simulink model "Pierre_Controller_LTI_2026b"  (R2025b)
settings: Solver=ode1  StartTime=0.0  StopTime=inf  FixedStep=Ts  RelTol=1e-3
PostLoadFcn:
  | , if any(exist('dsrtsu_mdlpostloadfcn', 'file') ~= 0), dsrtsu_mdlpostloadfcn('Execute', bdroot); end,
InitFcn:
  | , if any(exist('rtifpga_mdlclblib', 'file') ~= 0), rtifpga_mdlclblib('Init', bdroot); end,
values from neighbouring files (symbols this model uses):
  BUTTER = ss(A,B,C,D,Ts)    [build_model.m]
  K = opensave.K_final    [build_model.m]
  Px = 1    [build_model.m]
  Py = 1    [build_model.m]
  Pz = 1    [build_model.m]
  S_Sensor = 0.1134    [build_model.m]
  Sen_AX = 2.0176    [build_model.m]
  Sen_AY = 2.011    [build_model.m]
  Sen_AZ = 2.0066    [build_model.m]
  Sen_GX = 0.75481    [build_model.m]
  Sen_GY = 0.75728    [build_model.m]
  Sen_GZ = 0.74931    [build_model.m]
  Sweep_amp = 0.5    [build_model.m]
  Switch_excit = 4    [build_model.m]
  TMS_amp = 2    [build_model.m]
  TMS_freq1 = 80    [build_model.m]
  TMS_freq2 = 0    [build_model.m]
  TMS_freq3 = 0    [build_model.m]
  Ts = 1/Fs    (= 0.001)    [build_model.m]
  V_sat = 2/10    (= 0.2)    [build_model.m]
  V_sat_TMS = 5    [build_model.m]
undefined symbols (not defined in the file or in its folder): R, S
libraries: dspfdesign x15, rti1202lib_adc_class1 x10, rti1202lib_dac_class1 x7, rti1202lib_adc_class2 x6, dspxfrm3 x3, cstblocks x1, simulink x1
(part 1 of 3)
PreSaveFcn:
  | , if any(exist('dsmpb_private', 'file') == [2, 3, 6]), try, dsmpb_private('dsmpb_mdlclblib', 'PreSave', bdroot); catch, disp(lasterr); end, end,
CloseFcn:
  | , if any(exist('dsmpb_private', 'file') == [2, 3, 6]), try, dsmpb_private('dsmpb_mdlclblib', 'Close', bdroot); catch, disp(lasterr); end, end,
settings Model: DSRTSU_INTERNAL_RTI_VER=670  DSRTSU_INTERNAL_RTI_TYPE=rti1202  RTICANMMDATA=struct('GeneralSetupData',struct('modelroot','C:\PROJECTS\OSIP_VIB\Simulink\Feedback_LTI','generalsettings',struct('filesettings',struct('destfolder',struct('Name','RTICANMM_FILES','Check',1),'buildfolder',struct('Name','.','Check',1),'AbsDestfolder',struct('Name','C:\PROJECTS\OSIP_VIB\Simulink\Feedback_LTI\RTICANMM_FILES'),'AbsBuildfolder',struct('Name','C:\PROJECTS\OSIP_VIB\Simulink\Feedback_LTI'))),'options',struct('addpaths',1,'rmpaths',1,'addtrcexclusion',logical(1),'cannavigator',struct('checkmonitoring',0),'show_usrtrc',0,'use_usrtrc',0),'advanced',struct('options',[1 1 1 1 1 1 1 1 1 1 1 1 1 1 1 1 1 1 1 1 1 1 1 1 1 1 1 1 1 1 1 1 1 1 1 1 1 1 1 1 1 1 1 1 1 1 1 1 1 1 1 1 1 1 1 1 1 1 1 1 1 1 1 1 1 1 1 1 1 1 1 1 1 1 1 1 1 1 1 1 1 1 1 1 1 1 1 1 1 1 1 1 1 1 1 1 1 1 1 1]),'MPSetup',{{}},'modelname','Feedback_LTI','block','Feedback_LTI'))  DSRTSU_INTERNAL_RTIFPGA=231  DSMPB_DATASERVER_ModelPortLibVersion1=8  DSMPB_DATASERVER_DataServerVersion1=6  DSMPB_DATASERVER_DataServerStreamVersion1=3  DSRTSU_INTERNAL_RTISTBM_VER=25.2  Creator=yjr  LastModifiedBy=pgr
settings SolverCC: AlgebraicLoopSolver=TrustRegion
settings OptimizationCC: BlockReduction=off  OptimizeBlockIOStorage=off  BufferReuse=off  GlobalBufferReuse=off  ExpressionFolding=off  LocalBlockOutputs=off
settings DebuggingCC: UnconnectedInputMsg=warning  UnconnectedOutputMsg=warning  UnconnectedLineMsg=warning  ArithmeticOperatorsInVariantConditions=warning
settings HardwareCC: ProdBitPerPointer=32.0  ProdBitPerSizeT=32.0  ProdBitPerPtrDiffT=32.0  ProdLargestAtomicInteger=Integer  ProdEndianess=BigEndian  ProdWordSize=32.0  ProdHWDeviceType=Custom Processor->Custom  TargetIntDivRoundTo=Zero  TargetEndianess=BigEndian  TargetHWDeviceType=Custom Processor->Custom
settings ModelReferenceCC: EnableRefExpFcnMdlSchedulingChecks=on
settings SFSimCC: SimUseLocalCustomCode=off  MATLABDynamicMemAlloc=off  CustomCodeUndefinedFunction=UseInterfaceOnly
settings RTWCC: SystemTargetFile=rti1202.tlc  GenCodeOnly=on  MakeCommand=make_rti  TemplateMakefile=rti1202.tmf  RTWUseLocalCustomCode=off  GPUComputeCapability=3.5  Description=dSPACE DS1202 Hardware Platform
settings CodeAppCC: StateflowObjectComments=on
settings STFCustomTargetCC: SystemTargetFile=rti1202.tlc  ParMdlRefBuildCompliant=on  ConcurrentExecutionCompliant=off  GRTInterface=off  InitialSimState=RUN  LoadAfterBuild=off  TRCOnlyGlobals=off  EnableRealTimeTesting=on  BoardName=ds1202  TRCGenerateDerivatives=off  ExecutionMode=real-time  LoadApplNonUI=OFF  PlatformSelectionPopup=Platform Name  RTICfgSetVer=670.0  NISValue=1  NetworkClientNonUI=OPTION_DISABLED  TRCGenerateStates=off  CCompilerOptimizationOptsNonUI=USE_DEFAULT  TRCGenerateLabels=off  LoadToFlash=off  AllowReservedHostServiceNums=off  TimeScaleFactor=1.0  AssertionMode=OFF  TRCIsOmitVdOn=off  EnableRealTimeTestingNonUI=ON  ExecutionModeNonUI=RTSIM  VDFType=TRC  CCompilerOptimizationOptsPopup_=Default  FSIValue=0  TaskModeNonUI=LOW_JITTER  TRCGenerateVirtualBlocks=off  BoardNameNonUI=ds1202  TimeScaleFactorNonUI=OPTION_DISABLED  TaskMode=Low jitter, low latency tasks  TRCGenerateParamValues=on
settings GRTTargetCC: TargetLangStandard=C89/C90 (ANSI)  CompOptLevelCompliant=off  ConcurrentExecutionCompliant=off  CombineOutputUpdateFcns=off  MatFileLogging=off  CPPClassGenCompliant=off  UseToolchainInfoCompliant=off
settings ConfigComp: CovMetricSettings=dswe

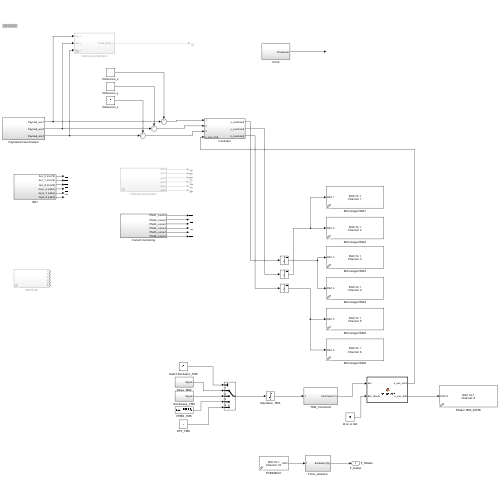
[thumbnail: Simulink's stored preview of the top-level diagram]
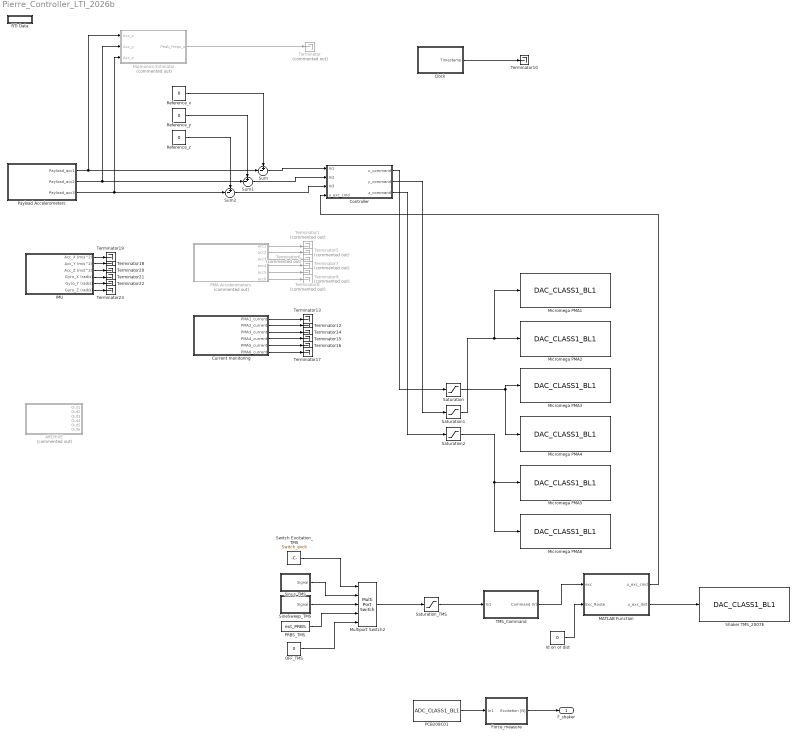
== system Pierre_Controller_LTI_2026b ==
  ARCHIVE : Subsystem  Commented=on
  Clock : Subsystem
  Controller : Subsystem
  Current monitoring : Subsystem
  Force_measure : Subsystem
  Harmonics Estimator : Subsystem  Commented=on
  IMU : Subsystem
  Id on or dist : Constant  Value=0
  MATLAB Function : MATLAB Function  TreatAsAtomicUnit=on
  Micromega PMA1 : rti1202lib_dac_class1/DAC_CLASS1_BL1  DSProperties=struct('RTI',struct('Version',uint32(2),'BlockType',struct('isSLSource',uint8(0),'isSLSink',uint8(1),'isHWSource',uint8(0),'isHWSink',uint8(1),'isSetup',uint8(0),'isInline',uint8(1),'isNonInline',uint8(0),'isInterrupt',uint8(0),'isChannelwise',uint8(1)),'IOBoardType',{{'DS120X','STD','DACC1'}},'UnitType','DAC','Identifier','DAC','DialogType','ML','BlockSet','NONE','SlaveProcessor','NONE'))  RTIBlockInterface=struct('InputPortsActive',1,'InputPortsWidth',int32(1),'InputPortsDataType',{{'SS_DOUBLE'}},'InputPortsName',{{['DAC 1']}},'DialogFcn','rti120xstddacc1dacgui','InitLevel',3,'IconTransparency','on','BlockDisplay',{{['DAC CL1\nChannel: 1'],'center'}},'BlockName',struct('Token',{{'DAC_CLASS1_BL1'}}))  RTIBlockParameters=struct('ChannelNo',{{1,'OFF',[]}},'ChannelNumOf',{{1,'OFF',[]}},'InitialValue1',{{0,'OFF',[-10 10]}},'InitialValue2',{{0,'OFF',[-10 10]}},'InitialValue3',{{0,'OFF',[-10 10]}},'InitialValue4',{{0,'OFF',[-10 10]}},'InitialValue5',{{0,'OFF',[-10 10]}},'InitialValue6',{{0,'OFF',[-10 10]}},'InitialValue7',{{0,'OFF',[-10 10]}},'InitialValue8',{{0,'OFF',[-10 10]}},'InitialValue9',{{0,'OFF',[-10 10]}},'InitialValue10',{{0,'OFF',[-10 10]}},'InitialValue11',{{0,'OFF',[-10 10]}},'InitialValue12',{{0,'OFF',[-10 10]}},'InitialValue13',{{0,'OFF',[-10 10]}},'InitialValue14',{{0,'OFF',[-10 10]}},'InitialValue15',{{0,'OFF',[-10 10]}},'InitialValue16',{{0,'OFF',[-10 10]}},'OutputMode',{{ones(1,16),'OFF',[1 2]}},'TermValue1',{{0,'OFF',[-10 10]}},'TermValue2',{{0,'OFF',[-10 10]}},'TermValue3',{{0,'OFF',[-10 10]}},'TermValue4',{{0,'OFF',[-10 10]}},'TermValue5',{{0,'OFF',[-10 10]}},'TermValue6',{{0,'OFF',[-10 10]}},'TermValue7',{{0,'OFF',[-10 10]}},'TermValue8',{{0,'OFF',[-10 10]}},'TermValue9',{{0,'OFF',[-10 10]}},'TermValue10',{{0,'OFF',[-10 10]}},'TermValue11',{{0,'OFF',[-10 10]}},'TermValue12',{{0,'OFF',[-10 10]}},'TermValue13',{{0,'OFF',[-10 10]}},'TermValue14',{{0,'OFF',[-10 10]}},'TermValue15',{{0,'OFF',[-10 10]}},'TermValue16',{{0,'OFF',[-10 10]}},'EnableTermMode',{{0,'OFF',[0 1]}},'TLCFileName',{{'rti120xdac_c1_dac','OFF',[]}},'InitialValueBuildCheck1',{{0,'OFF',[]}},'InitialValueBuildCheck2',{{0,'OFF',[]}},'InitialValueBuildCheck3',{{0,'OFF',[]}},'InitialValueBuildCheck4',{{0,'OFF',[]}},'InitialValueBuildCheck5',{{0,'OFF',[]}},'InitialValueBuildCheck6',{{0,'OFF',[]}},'InitialValueBuildCheck7',{{0,'OFF',[]}},'InitialValueBuildCheck8',{{0,'OFF',[]}},'InitialValueBuildCheck9',{{0,'OFF',[]}},'InitialValueBuildCheck10',{{0,'OFF',[]}},'InitialValueBuildCheck11',{{0,'OFF',[]}},'InitialValueBuildCheck12',{{0,'OFF',[]}},'InitialValueBuildCheck13',{{0,'OFF',[]}},'InitialValueBuildCheck14',{{0,'OFF',[]}},'InitialValueBuildCheck15',{{0,'OFF',[]}},'InitialValueBuildCheck16',{{0,'OFF',[]}},'TermValueBuildCheck1',{{0,'OFF',[]}},'TermValueBuildCheck2',{{0,'OFF',[]}},'TermValueBuildCheck3',{{0,'OFF',[]}},'TermValueBuildCheck4',{{0,'OFF',[]}},'TermValueBuildCheck5',{{0,'OFF',[]}},'TermValueBuildCheck6',{{0,'OFF',[]}},'TermValueBuildCheck7',{{0,'OFF',[]}},'TermValueBuildCheck8',{{0,'OFF',[]}},'TermValueBuildCheck9',{{0,'OFF',[]}},'TermValueBuildCheck10',{{0,'OFF',[]}},'TermValueBuildCheck11',{{0,'OFF',[]}},'TermValueBuildCheck12',{{0,'OFF',[]}},'TermValueBuildCheck13',{{0,'OFF',[]}},'TermValueBuildCheck14',{{0,'OFF',[]}},'TermValueBuildCheck15',{{0,'OFF',[]}},'TermValueBuildCheck16',{{0,'OFF',[]}})  RTISFcnParameters=struct('ChannelNo','int16','ChannelNumOf','int16','InitialValue1','double','InitialValue2','double','InitialValue3','double','InitialValue4','double','InitialValue5','double','InitialValue6','double','InitialValue7','double','InitialValue8','double','InitialValue9','double','InitialValue10','double','InitialValue11','double','InitialValue12','double','InitialValue13','double','InitialValue14','double','InitialValue15','double','InitialValue16','double','OutputMode','int16','TermValue1','double','TermValue2','double','TermValue3','double','TermValue4','double','TermValue5','double','TermValue6','double','TermValue7','double','TermValue8','double','TermValue9','double','TermValue10','double','TermValue11','double','TermValue12','double','TermValue13','double','TermValue14','double','TermValue15','double','TermValue16','double','EnableTermMode','int16','TLCFileName','char')  RTIBlockParaDefault=struct('ChannelNo',1,'ChannelNumOf',1,'InitialValue1',0,'InitialValue2',0,'InitialValue3',0,'InitialValue4',0,'InitialValue5',0,'InitialValue6',0,'InitialValue7',0,'InitialValue8',0,'InitialValue9',0,'InitialValue10',0,'InitialValue11',0,'InitialValue12',0,'InitialValue13',0,'InitialValue14',0,'InitialValue15',0,'InitialValue16',0,'OutputMode',ones(1,16),'TermValue1',0,'TermValue2',0,'TermValue3',0,'TermValue4',0,'TermValue5',0,'TermValue6',0,'TermValue7',0,'TermValue8',0,'TermValue9',0,'TermValue10',0,'TermValue11',0,'TermValue12',0,'TermValue13',0,'TermValue14',0,'TermValue15',0,'TermValue16',0,'EnableTermMode',0,'TLCFileName','rti120xdac_c1_dac','InitialValueBuildCheck1',0,'InitialValueBuildCheck2',0,'InitialValueBuildCheck3',0,'InitialValueBuildCheck4',0,'InitialValueBuildCheck5',0,'InitialValueBuildCheck6',0,'InitialValueBuildCheck7',0,'InitialValueBuildCheck8',0,'InitialValueBuildCheck9',0,'InitialValueBuildCheck10',0,'InitialValueBuildCheck11',0,'InitialValueBuildCheck12',0,'InitialValueBuildCheck13',0,'InitialValueBuildCheck14',0,'InitialValueBuildCheck15',0,'InitialValueBuildCheck16',0,'TermValueBuildCheck1',0,'TermValueBuildCheck2',0,'TermValueBuildCheck3',0,'TermValueBuildCheck4',0,'TermValueBuildCheck5',0,'TermValueBuildCheck6',0,'TermValueBuildCheck7',0,'TermValueBuildCheck8',0,'TermValueBuildCheck9',0,'TermValueBuildCheck10',0,'TermValueBuildCheck11',0,'TermValueBuildCheck12',0,'TermValueBuildCheck13',0,'TermValueBuildCheck14',0,'TermValueBuildCheck15',0,'TermValueBuildCheck16',0)
  Micromega PMA2 : rti1202lib_dac_class1/DAC_CLASS1_BL1  DSProperties=struct('RTI',struct('Version',uint32(2),'BlockType',struct('isSLSource',uint8(0),'isSLSink',uint8(1),'isHWSource',uint8(0),'isHWSink',uint8(1),'isSetup',uint8(0),'isInline',uint8(1),'isNonInline',uint8(0),'isInterrupt',uint8(0),'isChannelwise',uint8(1)),'IOBoardType',{{'DS120X','STD','DACC1'}},'UnitType','DAC','Identifier','DAC','DialogType','ML','BlockSet','NONE','SlaveProcessor','NONE'))  RTIBlockInterface=struct('InputPortsActive',1,'InputPortsWidth',int32(1),'InputPortsDataType',{{'SS_DOUBLE'}},'InputPortsName',{{['DAC 2']}},'DialogFcn','rti120xstddacc1dacgui','InitLevel',3,'IconTransparency','on','BlockDisplay',{{['DAC CL1\nChannel: 2'],'center'}},'BlockName',struct('Token',{{'DAC_CLASS1_BL1'}}))  RTIBlockParameters=struct('ChannelNo',{{2,'OFF',[]}},'ChannelNumOf',{{1,'OFF',[]}},'InitialValue1',{{'0','OFF',[-10 10]}},'InitialValue2',{{'0','OFF',[-10 10]}},'InitialValue3',{{'0','OFF',[-10 10]}},'InitialValue4',{{'0','OFF',[-10 10]}},'InitialValue5',{{'0','OFF',[-10 10]}},'InitialValue6',{{'0','OFF',[-10 10]}},'InitialValue7',{{'0','OFF',[-10 10]}},'InitialValue8',{{'0','OFF',[-10 10]}},'InitialValue9',{{'0','OFF',[-10 10]}},'InitialValue10',{{'0','OFF',[-10 10]}},'InitialValue11',{{'0','OFF',[-10 10]}},'InitialValue12',{{'0','OFF',[-10 10]}},'InitialValue13',{{'0','OFF',[-10 10]}},'InitialValue14',{{'0','OFF',[-10 10]}},'InitialValue15',{{'0','OFF',[-10 10]}},'InitialValue16',{{'0','OFF',[-10 10]}},'OutputMode',{{ones(1,16),'OFF',[1 2]}},'TermValue1',{{'0','OFF',[-10 10]}},'TermValue2',{{'0','OFF',[-10 10]}},'TermValue3',{{'0','OFF',[-10 10]}},'TermValue4',{{'0','OFF',[-10 10]}},'TermValue5',{{'0','OFF',[-10 10]}},'TermValue6',{{'0','OFF',[-10 10]}},'TermValue7',{{'0','OFF',[-10 10]}},'TermValue8',{{'0','OFF',[-10 10]}},'TermValue9',{{'0','OFF',[-10 10]}},'TermValue10',{{'0','OFF',[-10 10]}},'TermValue11',{{'0','OFF',[-10 10]}},'TermValue12',{{'0','OFF',[-10 10]}},'TermValue13',{{'0','OFF',[-10 10]}},'TermValue14',{{'0','OFF',[-10 10]}},'TermValue15',{{'0','OFF',[-10 10]}},'TermValue16',{{'0','OFF',[-10 10]}},'EnableTermMode',{{0,'OFF',[0 1]}},'TLCFileName',{{'rti120xdac_c1_dac','OFF',[]}},'InitialValueBuildCheck1',{{0,'OFF',[]}},'InitialValueBuildCheck2',{{1,'OFF',[]}},'InitialValueBuildCheck3',{{0,'OFF',[]}},'InitialValueBuildCheck4',{{0,'OFF',[]}},'InitialValueBuildCheck5',{{0,'OFF',[]}},'InitialValueBuildCheck6',{{0,'OFF',[]}},'InitialValueBuildCheck7',{{0,'OFF',[]}},'InitialValueBuildCheck8',{{0,'OFF',[]}},'InitialValueBuildCheck9',{{0,'OFF',[]}},'InitialValueBuildCheck10',{{0,'OFF',[]}},'InitialValueBuildCheck11',{{0,'OFF',[]}},'InitialValueBuildCheck12',{{0,'OFF',[]}},'InitialValueBuildCheck13',{{0,'OFF',[]}},'InitialValueBuildCheck14',{{0,'OFF',[]}},'InitialValueBuildCheck15',{{0,'OFF',[]}},'InitialValueBuildCheck16',{{0,'OFF',[]}},'TermValueBuildCheck1',{{0,'OFF',[]}},'TermValueBuildCheck2',{{0,'OFF',[]}},'TermValueBuildCheck3',{{0,'OFF',[]}},'TermValueBuildCheck4',{{0,'OFF',[]}},'TermValueBuildCheck5',{{0,'OFF',[]}},'TermValueBuildCheck6',{{0,'OFF',[]}},'TermValueBuildCheck7',{{0,'OFF',[]}},'TermValueBuildCheck8',{{0,'OFF',[]}},'TermValueBuildCheck9',{{0,'OFF',[]}},'TermValueBuildCheck10',{{0,'OFF',[]}},'TermValueBuildCheck11',{{0,'OFF',[]}},'TermValueBuildCheck12',{{0,'OFF',[]}},'TermValueBuildCheck13',{{0,'OFF',[]}},'TermValueBuildCheck14',{{0,'OFF',[]}},'TermValueBuildCheck15',{{0,'OFF',[]}},'TermValueBuildCheck16',{{0,'OFF',[]}})  RTISFcnParameters=struct('ChannelNo','int16','ChannelNumOf','int16','InitialValue1','double','InitialValue2','double','InitialValue3','double','InitialValue4','double','InitialValue5','double','InitialValue6','double','InitialValue7','double','InitialValue8','double','InitialValue9','double','InitialValue10','double','InitialValue11','double','InitialValue12','double','InitialValue13','double','InitialValue14','double','InitialValue15','double','InitialValue16','double','OutputMode','int16','TermValue1','double','TermValue2','double','TermValue3','double','TermValue4','double','TermValue5','double','TermValue6','double','TermValue7','double','TermValue8','double','TermValue9','double','TermValue10','double','TermValue11','double','TermValue12','double','TermValue13','double','TermValue14','double','TermValue15','double','TermValue16','double','EnableTermMode','int16','TLCFileName','char')  RTIBlockParaDefault=struct('ChannelNo',1,'ChannelNumOf',1,'InitialValue1',0,'InitialValue2',0,'InitialValue3',0,'InitialValue4',0,'InitialValue5',0,'InitialValue6',0,'InitialValue7',0,'InitialValue8',0,'InitialValue9',0,'InitialValue10',0,'InitialValue11',0,'InitialValue12',0,'InitialValue13',0,'InitialValue14',0,'InitialValue15',0,'InitialValue16',0,'OutputMode',ones(1,16),'TermValue1',0,'TermValue2',0,'TermValue3',0,'TermValue4',0,'TermValue5',0,'TermValue6',0,'TermValue7',0,'TermValue8',0,'TermValue9',0,'TermValue10',0,'TermValue11',0,'TermValue12',0,'TermValue13',0,'TermValue14',0,'TermValue15',0,'TermValue16',0,'EnableTermMode',0,'TLCFileName','rti120xdac_c1_dac','InitialValueBuildCheck1',0,'InitialValueBuildCheck2',0,'InitialValueBuildCheck3',0,'InitialValueBuildCheck4',0,'InitialValueBuildCheck5',0,'InitialValueBuildCheck6',0,'InitialValueBuildCheck7',0,'InitialValueBuildCheck8',0,'InitialValueBuildCheck9',0,'InitialValueBuildCheck10',0,'InitialValueBuildCheck11',0,'InitialValueBuildCheck12',0,'InitialValueBuildCheck13',0,'InitialValueBuildCheck14',0,'InitialValueBuildCheck15',0,'InitialValueBuildCheck16',0,'TermValueBuildCheck1',0,'TermValueBuildCheck2',0,'TermValueBuildCheck3',0,'TermValueBuildCheck4',0,'TermValueBuildCheck5',0,'TermValueBuildCheck6',0,'TermValueBuildCheck7',0,'TermValueBuildCheck8',0,'TermValueBuildCheck9',0,'TermValueBuildCheck10',0,'TermValueBuildCheck11',0,'TermValueBuildCheck12',0,'TermValueBuildCheck13',0,'TermValueBuildCheck14',0,'TermValueBuildCheck15',0,'TermValueBuildCheck16',0)
  Micromega PMA3 : rti1202lib_dac_class1/DAC_CLASS1_BL1  DSProperties=struct('RTI',struct('Version',uint32(2),'BlockType',struct('isSLSource',uint8(0),'isSLSink',uint8(1),'isHWSource',uint8(0),'isHWSink',uint8(1),'isSetup',uint8(0),'isInline',uint8(1),'isNonInline',uint8(0),'isInterrupt',uint8(0),'isChannelwise',uint8(1)),'IOBoardType',{{'DS120X','STD','DACC1'}},'UnitType','DAC','Identifier','DAC','DialogType','ML','BlockSet','NONE','SlaveProcessor','NONE'))  RTIBlockInterface=struct('InputPortsActive',1,'InputPortsWidth',int32(1),'InputPortsDataType',{{'SS_DOUBLE'}},'InputPortsName',{{['DAC 3']}},'DialogFcn','rti120xstddacc1dacgui','InitLevel',3,'IconTransparency','on','BlockDisplay',{{['DAC CL1\nChannel: 3'],'center'}},'BlockName',struct('Token',{{'DAC_CLASS1_BL1'}}))  RTIBlockParameters=struct('ChannelNo',{{3,'OFF',[]}},'ChannelNumOf',{{1,'OFF',[]}},'InitialValue1',{{'0','OFF',[-10 10]}},'InitialValue2',{{'0','OFF',[-10 10]}},'InitialValue3',{{'0','OFF',[-10 10]}},'InitialValue4',{{'0','OFF',[-10 10]}},'InitialValue5',{{'0','OFF',[-10 10]}},'InitialValue6',{{'0','OFF',[-10 10]}},'InitialValue7',{{'0','OFF',[-10 10]}},'InitialValue8',{{'0','OFF',[-10 10]}},'InitialValue9',{{'0','OFF',[-10 10]}},'InitialValue10',{{'0','OFF',[-10 10]}},'InitialValue11',{{'0','OFF',[-10 10]}},'InitialValue12',{{'0','OFF',[-10 10]}},'InitialValue13',{{'0','OFF',[-10 10]}},'InitialValue14',{{'0','OFF',[-10 10]}},'InitialValue15',{{'0','OFF',[-10 10]}},'InitialValue16',{{'0','OFF',[-10 10]}},'OutputMode',{{ones(1,16),'OFF',[1 2]}},'TermValue1',{{'0','OFF',[-10 10]}},'TermValue2',{{'0','OFF',[-10 10]}},'TermValue3',{{'0','OFF',[-10 10]}},'TermValue4',{{'0','OFF',[-10 10]}},'TermValue5',{{'0','OFF',[-10 10]}},'TermValue6',{{'0','OFF',[-10 10]}},'TermValue7',{{'0','OFF',[-10 10]}},'TermValue8',{{'0','OFF',[-10 10]}},'TermValue9',{{'0','OFF',[-10 10]}},'TermValue10',{{'0','OFF',[-10 10]}},'TermValue11',{{'0','OFF',[-10 10]}},'TermValue12',{{'0','OFF',[-10 10]}},'TermValue13',{{'0','OFF',[-10 10]}},'TermValue14',{{'0','OFF',[-10 10]}},'TermValue15',{{'0','OFF',[-10 10]}},'TermValue16',{{'0','OFF',[-10 10]}},'EnableTermMode',{{0,'OFF',[0 1]}},'TLCFileName',{{'rti120xdac_c1_dac','OFF',[]}},'InitialValueBuildCheck1',{{0,'OFF',[]}},'InitialValueBuildCheck2',{{0,'OFF',[]}},'InitialValueBuildCheck3',{{1,'OFF',[]}},'InitialValueBuildCheck4',{{0,'OFF',[]}},'InitialValueBuildCheck5',{{0,'OFF',[]}},'InitialValueBuildCheck6',{{0,'OFF',[]}},'InitialValueBuildCheck7',{{0,'OFF',[]}},'InitialValueBuildCheck8',{{0,'OFF',[]}},'InitialValueBuildCheck9',{{0,'OFF',[]}},'InitialValueBuildCheck10',{{0,'OFF',[]}},'InitialValueBuildCheck11',{{0,'OFF',[]}},'InitialValueBuildCheck12',{{0,'OFF',[]}},'InitialValueBuildCheck13',{{0,'OFF',[]}},'InitialValueBuildCheck14',{{0,'OFF',[]}},'InitialValueBuildCheck15',{{0,'OFF',[]}},'InitialValueBuildCheck16',{{0,'OFF',[]}},'TermValueBuildCheck1',{{0,'OFF',[]}},'TermValueBuildCheck2',{{0,'OFF',[]}},'TermValueBuildCheck3',{{0,'OFF',[]}},'TermValueBuildCheck4',{{0,'OFF',[]}},'TermValueBuildCheck5',{{0,'OFF',[]}},'TermValueBuildCheck6',{{0,'OFF',[]}},'TermValueBuildCheck7',{{0,'OFF',[]}},'TermValueBuildCheck8',{{0,'OFF',[]}},'TermValueBuildCheck9',{{0,'OFF',[]}},'TermValueBuildCheck10',{{0,'OFF',[]}},'TermValueBuildCheck11',{{0,'OFF',[]}},'TermValueBuildCheck12',{{0,'OFF',[]}},'TermValueBuildCheck13',{{0,'OFF',[]}},'TermValueBuildCheck14',{{0,'OFF',[]}},'TermValueBuildCheck15',{{0,'OFF',[]}},'TermValueBuildCheck16',{{0,'OFF',[]}})  RTISFcnParameters=struct('ChannelNo','int16','ChannelNumOf','int16','InitialValue1','double','InitialValue2','double','InitialValue3','double','InitialValue4','double','InitialValue5','double','InitialValue6','double','InitialValue7','double','InitialValue8','double','InitialValue9','double','InitialValue10','double','InitialValue11','double','InitialValue12','double','InitialValue13','double','InitialValue14','double','InitialValue15','double','InitialValue16','double','OutputMode','int16','TermValue1','double','TermValue2','double','TermValue3','double','TermValue4','double','TermValue5','double','TermValue6','double','TermValue7','double','TermValue8','double','TermValue9','double','TermValue10','double','TermValue11','double','TermValue12','double','TermValue13','double','TermValue14','double','TermValue15','double','TermValue16','double','EnableTermMode','int16','TLCFileName','char')  RTIBlockParaDefault=struct('ChannelNo',1,'ChannelNumOf',1,'InitialValue1',0,'InitialValue2',0,'InitialValue3',0,'InitialValue4',0,'InitialValue5',0,'InitialValue6',0,'InitialValue7',0,'InitialValue8',0,'InitialValue9',0,'InitialValue10',0,'InitialValue11',0,'InitialValue12',0,'InitialValue13',0,'InitialValue14',0,'InitialValue15',0,'InitialValue16',0,'OutputMode',ones(1,16),'TermValue1',0,'TermValue2',0,'TermValue3',0,'TermValue4',0,'TermValue5',0,'TermValue6',0,'TermValue7',0,'TermValue8',0,'TermValue9',0,'TermValue10',0,'TermValue11',0,'TermValue12',0,'TermValue13',0,'TermValue14',0,'TermValue15',0,'TermValue16',0,'EnableTermMode',0,'TLCFileName','rti120xdac_c1_dac','InitialValueBuildCheck1',0,'InitialValueBuildCheck2',0,'InitialValueBuildCheck3',0,'InitialValueBuildCheck4',0,'InitialValueBuildCheck5',0,'InitialValueBuildCheck6',0,'InitialValueBuildCheck7',0,'InitialValueBuildCheck8',0,'InitialValueBuildCheck9',0,'InitialValueBuildCheck10',0,'InitialValueBuildCheck11',0,'InitialValueBuildCheck12',0,'InitialValueBuildCheck13',0,'InitialValueBuildCheck14',0,'InitialValueBuildCheck15',0,'InitialValueBuildCheck16',0,'TermValueBuildCheck1',0,'TermValueBuildCheck2',0,'TermValueBuildCheck3',0,'TermValueBuildCheck4',0,'TermValueBuildCheck5',0,'TermValueBuildCheck6',0,'TermValueBuildCheck7',0,'TermValueBuildCheck8',0,'TermValueBuildCheck9',0,'TermValueBuildCheck10',0,'TermValueBuildCheck11',0,'TermValueBuildCheck12',0,'TermValueBuildCheck13',0,'TermValueBuildCheck14',0,'TermValueBuildCheck15',0,'TermValueBuildCheck16',0)
  Micromega PMA4 : rti1202lib_dac_class1/DAC_CLASS1_BL1  DSProperties=struct('RTI',struct('Version',uint32(2),'BlockType',struct('isSLSource',uint8(0),'isSLSink',uint8(1),'isHWSource',uint8(0),'isHWSink',uint8(1),'isSetup',uint8(0),'isInline',uint8(1),'isNonInline',uint8(0),'isInterrupt',uint8(0),'isChannelwise',uint8(1)),'IOBoardType',{{'DS120X','STD','DACC1'}},'UnitType','DAC','Identifier','DAC','DialogType','ML','BlockSet','NONE','SlaveProcessor','NONE'))  RTIBlockInterface=struct('InputPortsActive',1,'InputPortsWidth',int32(1),'InputPortsDataType',{{'SS_DOUBLE'}},'InputPortsName',{{['DAC 4']}},'DialogFcn','rti120xstddacc1dacgui','InitLevel',3,'IconTransparency','on','BlockDisplay',{{['DAC CL1\nChannel: 4'],'center'}},'BlockName',struct('Token',{{'DAC_CLASS1_BL1'}}))  RTIBlockParameters=struct('ChannelNo',{{4,'OFF',[]}},'ChannelNumOf',{{1,'OFF',[]}},'InitialValue1',{{'0','OFF',[-10 10]}},'InitialValue2',{{'0','OFF',[-10 10]}},'InitialValue3',{{'0','OFF',[-10 10]}},'InitialValue4',{{'0','OFF',[-10 10]}},'InitialValue5',{{'0','OFF',[-10 10]}},'InitialValue6',{{'0','OFF',[-10 10]}},'InitialValue7',{{'0','OFF',[-10 10]}},'InitialValue8',{{'0','OFF',[-10 10]}},'InitialValue9',{{'0','OFF',[-10 10]}},'InitialValue10',{{'0','OFF',[-10 10]}},'InitialValue11',{{'0','OFF',[-10 10]}},'InitialValue12',{{'0','OFF',[-10 10]}},'InitialValue13',{{'0','OFF',[-10 10]}},'InitialValue14',{{'0','OFF',[-10 10]}},'InitialValue15',{{'0','OFF',[-10 10]}},'InitialValue16',{{'0','OFF',[-10 10]}},'OutputMode',{{ones(1,16),'OFF',[1 2]}},'TermValue1',{{'0','OFF',[-10 10]}},'TermValue2',{{'0','OFF',[-10 10]}},'TermValue3',{{'0','OFF',[-10 10]}},'TermValue4',{{'0','OFF',[-10 10]}},'TermValue5',{{'0','OFF',[-10 10]}},'TermValue6',{{'0','OFF',[-10 10]}},'TermValue7',{{'0','OFF',[-10 10]}},'TermValue8',{{'0','OFF',[-10 10]}},'TermValue9',{{'0','OFF',[-10 10]}},'TermValue10',{{'0','OFF',[-10 10]}},'TermValue11',{{'0','OFF',[-10 10]}},'TermValue12',{{'0','OFF',[-10 10]}},'TermValue13',{{'0','OFF',[-10 10]}},'TermValue14',{{'0','OFF',[-10 10]}},'TermValue15',{{'0','OFF',[-10 10]}},'TermValue16',{{'0','OFF',[-10 10]}},'EnableTermMode',{{0,'OFF',[0 1]}},'TLCFileName',{{'rti120xdac_c1_dac','OFF',[]}},'InitialValueBuildCheck1',{{0,'OFF',[]}},'InitialValueBuildCheck2',{{0,'OFF',[]}},'InitialValueBuildCheck3',{{0,'OFF',[]}},'InitialValueBuildCheck4',{{1,'OFF',[]}},'InitialValueBuildCheck5',{{0,'OFF',[]}},'InitialValueBuildCheck6',{{0,'OFF',[]}},'InitialValueBuildCheck7',{{0,'OFF',[]}},'InitialValueBuildCheck8',{{0,'OFF',[]}},'InitialValueBuildCheck9',{{0,'OFF',[]}},'InitialValueBuildCheck10',{{0,'OFF',[]}},'InitialValueBuildCheck11',{{0,'OFF',[]}},'InitialValueBuildCheck12',{{0,'OFF',[]}},'InitialValueBuildCheck13',{{0,'OFF',[]}},'InitialValueBuildCheck14',{{0,'OFF',[]}},'InitialValueBuildCheck15',{{0,'OFF',[]}},'InitialValueBuildCheck16',{{0,'OFF',[]}},'TermValueBuildCheck1',{{0,'OFF',[]}},'TermValueBuildCheck2',{{0,'OFF',[]}},'TermValueBuildCheck3',{{0,'OFF',[]}},'TermValueBuildCheck4',{{0,'OFF',[]}},'TermValueBuildCheck5',{{0,'OFF',[]}},'TermValueBuildCheck6',{{0,'OFF',[]}},'TermValueBuildCheck7',{{0,'OFF',[]}},'TermValueBuildCheck8',{{0,'OFF',[]}},'TermValueBuildCheck9',{{0,'OFF',[]}},'TermValueBuildCheck10',{{0,'OFF',[]}},'TermValueBuildCheck11',{{0,'OFF',[]}},'TermValueBuildCheck12',{{0,'OFF',[]}},'TermValueBuildCheck13',{{0,'OFF',[]}},'TermValueBuildCheck14',{{0,'OFF',[]}},'TermValueBuildCheck15',{{0,'OFF',[]}},'TermValueBuildCheck16',{{0,'OFF',[]}})  RTISFcnParameters=struct('ChannelNo','int16','ChannelNumOf','int16','InitialValue1','double','InitialValue2','double','InitialValue3','double','InitialValue4','double','InitialValue5','double','InitialValue6','double','InitialValue7','double','InitialValue8','double','InitialValue9','double','InitialValue10','double','InitialValue11','double','InitialValue12','double','InitialValue13','double','InitialValue14','double','InitialValue15','double','InitialValue16','double','OutputMode','int16','TermValue1','double','TermValue2','double','TermValue3','double','TermValue4','double','TermValue5','double','TermValue6','double','TermValue7','double','TermValue8','double','TermValue9','double','TermValue10','double','TermValue11','double','TermValue12','double','TermValue13','double','TermValue14','double','TermValue15','double','TermValue16','double','EnableTermMode','int16','TLCFileName','char')  RTIBlockParaDefault=struct('ChannelNo',1,'ChannelNumOf',1,'InitialValue1',0,'InitialValue2',0,'InitialValue3',0,'InitialValue4',0,'InitialValue5',0,'InitialValue6',0,'InitialValue7',0,'InitialValue8',0,'InitialValue9',0,'InitialValue10',0,'InitialValue11',0,'InitialValue12',0,'InitialValue13',0,'InitialValue14',0,'InitialValue15',0,'InitialValue16',0,'OutputMode',ones(1,16),'TermValue1',0,'TermValue2',0,'TermValue3',0,'TermValue4',0,'TermValue5',0,'TermValue6',0,'TermValue7',0,'TermValue8',0,'TermValue9',0,'TermValue10',0,'TermValue11',0,'TermValue12',0,'TermValue13',0,'TermValue14',0,'TermValue15',0,'TermValue16',0,'EnableTermMode',0,'TLCFileName','rti120xdac_c1_dac','InitialValueBuildCheck1',0,'InitialValueBuildCheck2',0,'InitialValueBuildCheck3',0,'InitialValueBuildCheck4',0,'InitialValueBuildCheck5',0,'InitialValueBuildCheck6',0,'InitialValueBuildCheck7',0,'InitialValueBuildCheck8',0,'InitialValueBuildCheck9',0,'InitialValueBuildCheck10',0,'InitialValueBuildCheck11',0,'InitialValueBuildCheck12',0,'InitialValueBuildCheck13',0,'InitialValueBuildCheck14',0,'InitialValueBuildCheck15',0,'InitialValueBuildCheck16',0,'TermValueBuildCheck1',0,'TermValueBuildCheck2',0,'TermValueBuildCheck3',0,'TermValueBuildCheck4',0,'TermValueBuildCheck5',0,'TermValueBuildCheck6',0,'TermValueBuildCheck7',0,'TermValueBuildCheck8',0,'TermValueBuildCheck9',0,'TermValueBuildCheck10',0,'TermValueBuildCheck11',0,'TermValueBuildCheck12',0,'TermValueBuildCheck13',0,'TermValueBuildCheck14',0,'TermValueBuildCheck15',0,'TermValueBuildCheck16',0)
  Micromega PMA5 : rti1202lib_dac_class1/DAC_CLASS1_BL1  DSProperties=struct('RTI',struct('Version',uint32(2),'BlockType',struct('isSLSource',uint8(0),'isSLSink',uint8(1),'isHWSource',uint8(0),'isHWSink',uint8(1),'isSetup',uint8(0),'isInline',uint8(1),'isNonInline',uint8(0),'isInterrupt',uint8(0),'isChannelwise',uint8(1)),'IOBoardType',{{'DS120X','STD','DACC1'}},'UnitType','DAC','Identifier','DAC','DialogType','ML','BlockSet','NONE','SlaveProcessor','NONE'))  RTIBlockInterface=struct('InputPortsActive',1,'InputPortsWidth',int32(1),'InputPortsDataType',{{'SS_DOUBLE'}},'InputPortsName',{{['DAC 5']}},'DialogFcn','rti120xstddacc1dacgui','InitLevel',3,'IconTransparency','on','BlockDisplay',{{['DAC CL1\nChannel: 5'],'center'}},'BlockName',struct('Token',{{'DAC_CLASS1_BL1'}}))  RTIBlockParameters=struct('ChannelNo',{{5,'OFF',[]}},'ChannelNumOf',{{1,'OFF',[]}},'InitialValue1',{{'0','OFF',[-10 10]}},'InitialValue2',{{'0','OFF',[-10 10]}},'InitialValue3',{{'0','OFF',[-10 10]}},'InitialValue4',{{'0','OFF',[-10 10]}},'InitialValue5',{{'0','OFF',[-10 10]}},'InitialValue6',{{'0','OFF',[-10 10]}},'InitialValue7',{{'0','OFF',[-10 10]}},'InitialValue8',{{'0','OFF',[-10 10]}},'InitialValue9',{{'0','OFF',[-10 10]}},'InitialValue10',{{'0','OFF',[-10 10]}},'InitialValue11',{{'0','OFF',[-10 10]}},'InitialValue12',{{'0','OFF',[-10 10]}},'InitialValue13',{{'0','OFF',[-10 10]}},'InitialValue14',{{'0','OFF',[-10 10]}},'InitialValue15',{{'0','OFF',[-10 10]}},'InitialValue16',{{'0','OFF',[-10 10]}},'OutputMode',{{ones(1,16),'OFF',[1 2]}},'TermValue1',{{'0','OFF',[-10 10]}},'TermValue2',{{'0','OFF',[-10 10]}},'TermValue3',{{'0','OFF',[-10 10]}},'TermValue4',{{'0','OFF',[-10 10]}},'TermValue5',{{'0','OFF',[-10 10]}},'TermValue6',{{'0','OFF',[-10 10]}},'TermValue7',{{'0','OFF',[-10 10]}},'TermValue8',{{'0','OFF',[-10 10]}},'TermValue9',{{'0','OFF',[-10 10]}},'TermValue10',{{'0','OFF',[-10 10]}},'TermValue11',{{'0','OFF',[-10 10]}},'TermValue12',{{'0','OFF',[-10 10]}},'TermValue13',{{'0','OFF',[-10 10]}},'TermValue14',{{'0','OFF',[-10 10]}},'TermValue15',{{'0','OFF',[-10 10]}},'TermValue16',{{'0','OFF',[-10 10]}},'EnableTermMode',{{0,'OFF',[0 1]}},'TLCFileName',{{'rti120xdac_c1_dac','OFF',[]}},'InitialValueBuildCheck1',{{0,'OFF',[]}},'InitialValueBuildCheck2',{{0,'OFF',[]}},'InitialValueBuildCheck3',{{0,'OFF',[]}},'InitialValueBuildCheck4',{{0,'OFF',[]}},'InitialValueBuildCheck5',{{1,'OFF',[]}},'InitialValueBuildCheck6',{{0,'OFF',[]}},'InitialValueBuildCheck7',{{0,'OFF',[]}},'InitialValueBuildCheck8',{{0,'OFF',[]}},'InitialValueBuildCheck9',{{0,'OFF',[]}},'InitialValueBuildCheck10',{{0,'OFF',[]}},'InitialValueBuildCheck11',{{0,'OFF',[]}},'InitialValueBuildCheck12',{{0,'OFF',[]}},'InitialValueBuildCheck13',{{0,'OFF',[]}},'InitialValueBuildCheck14',{{0,'OFF',[]}},'InitialValueBuildCheck15',{{0,'OFF',[]}},'InitialValueBuildCheck16',{{0,'OFF',[]}},'TermValueBuildCheck1',{{0,'OFF',[]}},'TermValueBuildCheck2',{{0,'OFF',[]}},'TermValueBuildCheck3',{{0,'OFF',[]}},'TermValueBuildCheck4',{{0,'OFF',[]}},'TermValueBuildCheck5',{{0,'OFF',[]}},'TermValueBuildCheck6',{{0,'OFF',[]}},'TermValueBuildCheck7',{{0,'OFF',[]}},'TermValueBuildCheck8',{{0,'OFF',[]}},'TermValueBuildCheck9',{{0,'OFF',[]}},'TermValueBuildCheck10',{{0,'OFF',[]}},'TermValueBuildCheck11',{{0,'OFF',[]}},'TermValueBuildCheck12',{{0,'OFF',[]}},'TermValueBuildCheck13',{{0,'OFF',[]}},'TermValueBuildCheck14',{{0,'OFF',[]}},'TermValueBuildCheck15',{{0,'OFF',[]}},'TermValueBuildCheck16',{{0,'OFF',[]}})  RTISFcnParameters=struct('ChannelNo','int16','ChannelNumOf','int16','InitialValue1','double','InitialValue2','double','InitialValue3','double','InitialValue4','double','InitialValue5','double','InitialValue6','double','InitialValue7','double','InitialValue8','double','InitialValue9','double','InitialValue10','double','InitialValue11','double','InitialValue12','double','InitialValue13','double','InitialValue14','double','InitialValue15','double','InitialValue16','double','OutputMode','int16','TermValue1','double','TermValue2','double','TermValue3','double','TermValue4','double','TermValue5','double','TermValue6','double','TermValue7','double','TermValue8','double','TermValue9','double','TermValue10','double','TermValue11','double','TermValue12','double','TermValue13','double','TermValue14','double','TermValue15','double','TermValue16','double','EnableTermMode','int16','TLCFileName','char')  RTIBlockParaDefault=struct('ChannelNo',1,'ChannelNumOf',1,'InitialValue1',0,'InitialValue2',0,'InitialValue3',0,'InitialValue4',0,'InitialValue5',0,'InitialValue6',0,'InitialValue7',0,'InitialValue8',0,'InitialValue9',0,'InitialValue10',0,'InitialValue11',0,'InitialValue12',0,'InitialValue13',0,'InitialValue14',0,'InitialValue15',0,'InitialValue16',0,'OutputMode',ones(1,16),'TermValue1',0,'TermValue2',0,'TermValue3',0,'TermValue4',0,'TermValue5',0,'TermValue6',0,'TermValue7',0,'TermValue8',0,'TermValue9',0,'TermValue10',0,'TermValue11',0,'TermValue12',0,'TermValue13',0,'TermValue14',0,'TermValue15',0,'TermValue16',0,'EnableTermMode',0,'TLCFileName','rti120xdac_c1_dac','InitialValueBuildCheck1',0,'InitialValueBuildCheck2',0,'InitialValueBuildCheck3',0,'InitialValueBuildCheck4',0,'InitialValueBuildCheck5',0,'InitialValueBuildCheck6',0,'InitialValueBuildCheck7',0,'InitialValueBuildCheck8',0,'InitialValueBuildCheck9',0,'InitialValueBuildCheck10',0,'InitialValueBuildCheck11',0,'InitialValueBuildCheck12',0,'InitialValueBuildCheck13',0,'InitialValueBuildCheck14',0,'InitialValueBuildCheck15',0,'InitialValueBuildCheck16',0,'TermValueBuildCheck1',0,'TermValueBuildCheck2',0,'TermValueBuildCheck3',0,'TermValueBuildCheck4',0,'TermValueBuildCheck5',0,'TermValueBuildCheck6',0,'TermValueBuildCheck7',0,'TermValueBuildCheck8',0,'TermValueBuildCheck9',0,'TermValueBuildCheck10',0,'TermValueBuildCheck11',0,'TermValueBuildCheck12',0,'TermValueBuildCheck13',0,'TermValueBuildCheck14',0,'TermValueBuildCheck15',0,'TermValueBuildCheck16',0)
  Micromega PMA6 : rti1202lib_dac_class1/DAC_CLASS1_BL1  DSProperties=struct('RTI',struct('Version',uint32(2),'BlockType',struct('isSLSource',uint8(0),'isSLSink',uint8(1),'isHWSource',uint8(0),'isHWSink',uint8(1),'isSetup',uint8(0),'isInline',uint8(1),'isNonInline',uint8(0),'isInterrupt',uint8(0),'isChannelwise',uint8(1)),'IOBoardType',{{'DS120X','STD','DACC1'}},'UnitType','DAC','Identifier','DAC','DialogType','ML','BlockSet','NONE','SlaveProcessor','NONE'))  RTIBlockInterface=struct('InputPortsActive',1,'InputPortsWidth',int32(1),'InputPortsDataType',{{'SS_DOUBLE'}},'InputPortsName',{{['DAC 6']}},'DialogFcn','rti120xstddacc1dacgui','InitLevel',3,'IconTransparency','on','BlockDisplay',{{['DAC CL1\nChannel: 6'],'center'}},'BlockName',struct('Token',{{'DAC_CLASS1_BL1'}}))  RTIBlockParameters=struct('ChannelNo',{{6,'OFF',[]}},'ChannelNumOf',{{1,'OFF',[]}},'InitialValue1',{{'0','OFF',[-10 10]}},'InitialValue2',{{'0','OFF',[-10 10]}},'InitialValue3',{{'0','OFF',[-10 10]}},'InitialValue4',{{'0','OFF',[-10 10]}},'InitialValue5',{{'0','OFF',[-10 10]}},'InitialValue6',{{'0','OFF',[-10 10]}},'InitialValue7',{{'0','OFF',[-10 10]}},'InitialValue8',{{'0','OFF',[-10 10]}},'InitialValue9',{{'0','OFF',[-10 10]}},'InitialValue10',{{'0','OFF',[-10 10]}},'InitialValue11',{{'0','OFF',[-10 10]}},'InitialValue12',{{'0','OFF',[-10 10]}},'InitialValue13',{{'0','OFF',[-10 10]}},'InitialValue14',{{'0','OFF',[-10 10]}},'InitialValue15',{{'0','OFF',[-10 10]}},'InitialValue16',{{'0','OFF',[-10 10]}},'OutputMode',{{ones(1,16),'OFF',[1 2]}},'TermValue1',{{'0','OFF',[-10 10]}},'TermValue2',{{'0','OFF',[-10 10]}},'TermValue3',{{'0','OFF',[-10 10]}},'TermValue4',{{'0','OFF',[-10 10]}},'TermValue5',{{'0','OFF',[-10 10]}},'TermValue6',{{'0','OFF',[-10 10]}},'TermValue7',{{'0','OFF',[-10 10]}},'TermValue8',{{'0','OFF',[-10 10]}},'TermValue9',{{'0','OFF',[-10 10]}},'TermValue10',{{'0','OFF',[-10 10]}},'TermValue11',{{'0','OFF',[-10 10]}},'TermValue12',{{'0','OFF',[-10 10]}},'TermValue13',{{'0','OFF',[-10 10]}},'TermValue14',{{'0','OFF',[-10 10]}},'TermValue15',{{'0','OFF',[-10 10]}},'TermValue16',{{'0','OFF',[-10 10]}},'EnableTermMode',{{0,'OFF',[0 1]}},'TLCFileName',{{'rti120xdac_c1_dac','OFF',[]}},'InitialValueBuildCheck1',{{0,'OFF',[]}},'InitialValueBuildCheck2',{{0,'OFF',[]}},'InitialValueBuildCheck3',{{0,'OFF',[]}},'InitialValueBuildCheck4',{{0,'OFF',[]}},'InitialValueBuildCheck5',{{0,'OFF',[]}},'InitialValueBuildCheck6',{{1,'OFF',[]}},'InitialValueBuildCheck7',{{0,'OFF',[]}},'InitialValueBuildCheck8',{{0,'OFF',[]}},'InitialValueBuildCheck9',{{0,'OFF',[]}},'InitialValueBuildCheck10',{{0,'OFF',[]}},'InitialValueBuildCheck11',{{0,'OFF',[]}},'InitialValueBuildCheck12',{{0,'OFF',[]}},'InitialValueBuildCheck13',{{0,'OFF',[]}},'InitialValueBuildCheck14',{{0,'OFF',[]}},'InitialValueBuildCheck15',{{0,'OFF',[]}},'InitialValueBuildCheck16',{{0,'OFF',[]}},'TermValueBuildCheck1',{{0,'OFF',[]}},'TermValueBuildCheck2',{{0,'OFF',[]}},'TermValueBuildCheck3',{{0,'OFF',[]}},'TermValueBuildCheck4',{{0,'OFF',[]}},'TermValueBuildCheck5',{{0,'OFF',[]}},'TermValueBuildCheck6',{{0,'OFF',[]}},'TermValueBuildCheck7',{{0,'OFF',[]}},'TermValueBuildCheck8',{{0,'OFF',[]}},'TermValueBuildCheck9',{{0,'OFF',[]}},'TermValueBuildCheck10',{{0,'OFF',[]}},'TermValueBuildCheck11',{{0,'OFF',[]}},'TermValueBuildCheck12',{{0,'OFF',[]}},'TermValueBuildCheck13',{{0,'OFF',[]}},'TermValueBuildCheck14',{{0,'OFF',[]}},'TermValueBuildCheck15',{{0,'OFF',[]}},'TermValueBuildCheck16',{{0,'OFF',[]}})  RTISFcnParameters=struct('ChannelNo','int16','ChannelNumOf','int16','InitialValue1','double','InitialValue2','double','InitialValue3','double','InitialValue4','double','InitialValue5','double','InitialValue6','double','InitialValue7','double','InitialValue8','double','InitialValue9','double','InitialValue10','double','InitialValue11','double','InitialValue12','double','InitialValue13','double','InitialValue14','double','InitialValue15','double','InitialValue16','double','OutputMode','int16','TermValue1','double','TermValue2','double','TermValue3','double','TermValue4','double','TermValue5','double','TermValue6','double','TermValue7','double','TermValue8','double','TermValue9','double','TermValue10','double','TermValue11','double','TermValue12','double','TermValue13','double','TermValue14','double','TermValue15','double','TermValue16','double','EnableTermMode','int16','TLCFileName','char')  RTIBlockParaDefault=struct('ChannelNo',1,'ChannelNumOf',1,'InitialValue1',0,'InitialValue2',0,'InitialValue3',0,'InitialValue4',0,'InitialValue5',0,'InitialValue6',0,'InitialValue7',0,'InitialValue8',0,'InitialValue9',0,'InitialValue10',0,'InitialValue11',0,'InitialValue12',0,'InitialValue13',0,'InitialValue14',0,'InitialValue15',0,'InitialValue16',0,'OutputMode',ones(1,16),'TermValue1',0,'TermValue2',0,'TermValue3',0,'TermValue4',0,'TermValue5',0,'TermValue6',0,'TermValue7',0,'TermValue8',0,'TermValue9',0,'TermValue10',0,'TermValue11',0,'TermValue12',0,'TermValue13',0,'TermValue14',0,'TermValue15',0,'TermValue16',0,'EnableTermMode',0,'TLCFileName','rti120xdac_c1_dac','InitialValueBuildCheck1',0,'InitialValueBuildCheck2',0,'InitialValueBuildCheck3',0,'InitialValueBuildCheck4',0,'InitialValueBuildCheck5',0,'InitialValueBuildCheck6',0,'InitialValueBuildCheck7',0,'InitialValueBuildCheck8',0,'InitialValueBuildCheck9',0,'InitialValueBuildCheck10',0,'InitialValueBuildCheck11',0,'InitialValueBuildCheck12',0,'InitialValueBuildCheck13',0,'InitialValueBuildCheck14',0,'InitialValueBuildCheck15',0,'InitialValueBuildCheck16',0,'TermValueBuildCheck1',0,'TermValueBuildCheck2',0,'TermValueBuildCheck3',0,'TermValueBuildCheck4',0,'TermValueBuildCheck5',0,'TermValueBuildCheck6',0,'TermValueBuildCheck7',0,'TermValueBuildCheck8',0,'TermValueBuildCheck9',0,'TermValueBuildCheck10',0,'TermValueBuildCheck11',0,'TermValueBuildCheck12',0,'TermValueBuildCheck13',0,'TermValueBuildCheck14',0,'TermValueBuildCheck15',0,'TermValueBuildCheck16',0)
  Multiport Switch2 : MultiPortSwitch  Inputs=4  DiagnosticForDefault=Warning  SaturateOnIntegerOverflow=off  InputSameDT=off
  OFF_TMS : Constant  Value=0
  PCB208C01 : rti1202lib_adc_class1/ADC_CLASS1_BL1  DSProperties=struct('RTI',struct('Version',uint32(1),'BlockType',struct('isSLSource',uint8(1),'isSLSink',uint8(1),'isHWSource',uint8(0),'isHWSink',uint8(1),'isSetup',uint8(0),'isInline',uint8(1),'isNonInline',uint8(0),'isInterrupt',uint8(0),'isChannelwise',uint8(1)),'IOBoardType',{{'DS120X','STD','ADCC1'}},'UnitType','ADC','Identifier','ADC','DialogType','ML','BlockSet','NONE','SlaveProcessor','NONE'))  RTIBlockInterface=struct('InputPortsActive',0,'InputPortsWidth',int32(1),'InputPortsDataType',{{'SS_BOOLEAN'}},'InputPortsName',{{'Continue'}},'OutputPortsActive',[1 0],'OutputPortsWidth',int32([1 1]),'OutputPortsDataType',{{'SS_DOUBLE','SS_INT16'}},'OutputPortsName',{{'ADC','Status'}},'DialogFcn','rti120xstdadcc1adcgui','SampleTime',{{-1}},'InitLevel',3,'IconTransparency','on','BlockDisplay',{{['ADC CL1\nChannel: 16'],'center'}},'BlockName',struct('Token',{{'ADC_CLASS1_BL1'}}))  RTIBlockParameters=struct('ReadMode',{{1,'OFF',[1 2]}},'ChannelNo',{{16,'OFF',[]}},'ConversionMode',{{1,'OFF',[1 2]}},'TriggerSource',{{1,'OFF',[1 2]}},'TriggerLineIn',{{1,'OFF',[1 16]}},'SampleMode',{{1,'OFF',[1 2]}},'BurstTriggerSource',{{1,'OFF',[1 2]}},'BurstTriggerLine',{{1,'OFF',[1 16]}},'ConvTriggerSource',{{3,'OFF',[1 3]}},'ConvTriggerLine',{{1,'OFF',[1 16]}},'ConvPeriod',{{'100e-6','OFF',[1e-6 1.34]}},'ConvPeriodCheck',{{0,'OFF',[]}},'BurstSize',{{'10','OFF',[]}},'BurstSizeCheck',{{0,'OFF',[]}},'DataSetOffset',{{'0','OFF',[]}},'DataSetOffsetCheck',{{0,'OFF',[]}},'DataSetLength',{{'1','OFF',[]}},'DataSetLengthCheck',{{0,'OFF',[]}},'EnableTriggerEvent',{{0,'OFF',[0 1]}},'TriggerMode',{{2,'OFF',[1 3]}},'TriggerLineOut',{{1,'OFF',[1 16]}},'ADCSWStartEnable',{{0,'OFF',[0 1]}},'SampleTime',{{'-1','OFF',[-1 inf]}},'SampleTimeCheck',{{1,'OFF',[]}},'StatusPortEnable',{{0,'OFF',[0 1]}},'TLCFileName',{{'rti120xadc_c1_adc','OFF',[]}})  RTISFcnParameters=struct('ReadMode','int16','ChannelNo','int16','ConversionMode','int16','TriggerSource','int16','TriggerLineIn','int16','SampleMode','int16','BurstTriggerSource','int16','BurstTriggerLine','int16','ConvTriggerSource','int16','ConvTriggerLine','int16','ConvPeriod','double','BurstSize','int16','DataSetOffset','int16','DataSetLength','int16','EnableTriggerEvent','int16','TriggerMode','int16','TriggerLineOut','int16','ADCSWStartEnable','int16','SampleTime','double','StatusPortEnable','int16','TLCFileName','char')  RTIBlockParaDefault=struct('ReadMode',1,'ChannelNo',1,'ConversionMode',1,'TriggerSource',1,'TriggerLineIn',1,'SampleMode',1,'BurstTriggerSource',1,'BurstTriggerLine',1,'ConvTriggerSource',3,'ConvTriggerLine',1,'ConvPeriod',0.0001,'ConvPeriodCheck',0,'BurstSize',10,'BurstSizeCheck',0,'DataSetOffset',0,'DataSetOffsetCheck',0,'DataSetLength',1,'DataSetLengthCheck',0,'EnableTriggerEvent',0,'TriggerMode',2,'TriggerLineOut',1,'ADCSWStartEnable',0,'SampleTime',-1,'SampleTimeCheck',1,'StatusPortEnable',0,'TLCFileName','rti120xadc_c1_adc')
  PMA Accelerometers : Subsystem  Commented=on
  PRBS_TMS : FromWorkspace  VariableName=ext_PRBS  SampleTime=Ts
  Payload Accelerometers : Subsystem
  RTI Data : Subsystem  Tag=struct('RTIDataServer',struct('RTIDataServerVs','2','RTIModelDescription','struct(''main'',''Pierre_Controller_LTI'',''sub'',''Pierre_Controller_LTI'',''isMp'',0)'))  LoadFcn="if exist('rtidc'), try,  rtidc('DataHostBlockClbLoad', gcbh); catch, disp(['Warning: ''LoadFcn'' for RTI Data block failed: ' lasterr]); end, end,"  mask(RTI_DATA_HOST){}
      mask help:
      | RTI Data Block.
      | This block is used by RTI to store internal model-dependent data.
      | Please keep this block on the root level of the model. Deleting this block will result in data loss.
      |
      | NEVER DELETE OR COPY THIS BLOCK!
      settings: CopyFcn="if exist('rtidc'), try,  rtidc('DataHostBlockClbCopy', gcbh); catch, disp(['Warning: ''CopyFcn'' for RTI Data block failed: ' lasterr]); end, end,"  DeleteFcn="if exist('rtidc'), try,  rtidc('DataHostBlockClbDelete', gcbh); catch, disp(['Warning: ''DeleteFcn'' for RTI Data block failed: ' lasterr]); end, end,"  ModelCloseFcn="if exist('rtidc'), try,  rtidc('DataHostBlockClbModelClose', gcbh); catch, disp(['Warning: ''ModelCloseFcn'' for RTI Data block failed: ' lasterr]); end, end,"  PreSaveFcn="if exist('rtidc'), try,  rtidc('DataHostBlockClbPreSave', gcbh); catch, disp(['Warning: ''PreSaveFcn'' for RTI Data block failed: ' lasterr]); end, end,"  PostSaveFcn="if exist('rtidc'), try,  rtidc('DataHostBlockClbPostSave', gcbh); catch, disp(['Warning: ''PostSaveFcn'' for RTI Data block failed: ' lasterr]); end, end,"  NameChangeFcn="if exist('rtidc'), try,  rtidc('DataHostBlockClbNameChange', gcbh); catch, disp(['Warning: ''NameChangeFcn'' for RTI Data block failed: ' lasterr]); end, end,"
      mask Help:
      | RTI Data Block.
      | This block is used by RTI to store internal model-dependent data.
      | Please keep this block on the root level of the model. Deleting this block will result in data loss.
      | 
      | NEVER DELETE OR COPY THIS BLOCK!
      mask Display:
      | text(0.5, 0.5, 'RTI Data', 'HorizontalAlignment', 'center');
      | plot([1 0]);
  Reference_x : Constant  Value=0  SampleTime=Ts
  Reference_y : Constant  Value=0  SampleTime=Ts
  Reference_z : Constant  Value=0  SampleTime=Ts
  Saturation : Saturate  UpperLimit=V_sat  LowerLimit=-V_sat
  Saturation1 : Saturate  UpperLimit=V_sat  LowerLimit=-V_sat
  Saturation2 : Saturate  UpperLimit=V_sat  LowerLimit=-V_sat
  Saturation_TMS : Saturate  UpperLimit=V_sat_TMS  LowerLimit=-V_sat_TMS
  Shaker TMS_2007E : rti1202lib_dac_class1/DAC_CLASS1_BL1  DSProperties=struct('RTI',struct('Version',uint32(2),'BlockType',struct('isSLSource',uint8(0),'isSLSink',uint8(1),'isHWSource',uint8(0),'isHWSink',uint8(1),'isSetup',uint8(0),'isInline',uint8(1),'isNonInline',uint8(0),'isInterrupt',uint8(0),'isChannelwise',uint8(1)),'IOBoardType',{{'DS120X','STD','DACC1'}},'UnitType','DAC','Identifier','DAC','DialogType','ML','BlockSet','NONE','SlaveProcessor','NONE'))  RTIBlockInterface=struct('InputPortsActive',1,'InputPortsWidth',int32(1),'InputPortsDataType',{{'SS_DOUBLE'}},'InputPortsName',{{['DAC 9']}},'DialogFcn','rti120xstddacc1dacgui','InitLevel',3,'IconTransparency','on','BlockDisplay',{{['DAC CL1\nChannel: 9'],'center'}},'BlockName',struct('Token',{{'DAC_CLASS1_BL1'}}))  RTIBlockParameters=struct('ChannelNo',{{9,'OFF',[]}},'ChannelNumOf',{{1,'OFF',[]}},'InitialValue1',{{'0','OFF',[-10 10]}},'InitialValue2',{{'0','OFF',[-10 10]}},'InitialValue3',{{'0','OFF',[-10 10]}},'InitialValue4',{{'0','OFF',[-10 10]}},'InitialValue5',{{'0','OFF',[-10 10]}},'InitialValue6',{{'0','OFF',[-10 10]}},'InitialValue7',{{'0','OFF',[-10 10]}},'InitialValue8',{{'0','OFF',[-10 10]}},'InitialValue9',{{'0','OFF',[-10 10]}},'InitialValue10',{{'0','OFF',[-10 10]}},'InitialValue11',{{'0','OFF',[-10 10]}},'InitialValue12',{{'0','OFF',[-10 10]}},'InitialValue13',{{'0','OFF',[-10 10]}},'InitialValue14',{{'0','OFF',[-10 10]}},'InitialValue15',{{'0','OFF',[-10 10]}},'InitialValue16',{{'0','OFF',[-10 10]}},'OutputMode',{{ones(1,16),'OFF',[1 2]}},'TermValue1',{{'0','OFF',[-10 10]}},'TermValue2',{{'0','OFF',[-10 10]}},'TermValue3',{{'0','OFF',[-10 10]}},'TermValue4',{{'0','OFF',[-10 10]}},'TermValue5',{{'0','OFF',[-10 10]}},'TermValue6',{{'0','OFF',[-10 10]}},'TermValue7',{{'0','OFF',[-10 10]}},'TermValue8',{{'0','OFF',[-10 10]}},'TermValue9',{{'0','OFF',[-10 10]}},'TermValue10',{{'0','OFF',[-10 10]}},'TermValue11',{{'0','OFF',[-10 10]}},'TermValue12',{{'0','OFF',[-10 10]}},'TermValue13',{{'0','OFF',[-10 10]}},'TermValue14',{{'0','OFF',[-10 10]}},'TermValue15',{{'0','OFF',[-10 10]}},'TermValue16',{{'0','OFF',[-10 10]}},'EnableTermMode',{{0,'OFF',[0 1]}},'TLCFileName',{{'rti120xdac_c1_dac','OFF',[]}},'InitialValueBuildCheck1',{{0,'OFF',[]}},'InitialValueBuildCheck2',{{0,'OFF',[]}},'InitialValueBuildCheck3',{{0,'OFF',[]}},'InitialValueBuildCheck4',{{0,'OFF',[]}},'InitialValueBuildCheck5',{{0,'OFF',[]}},'InitialValueBuildCheck6',{{0,'OFF',[]}},'InitialValueBuildCheck7',{{0,'OFF',[]}},'InitialValueBuildCheck8',{{0,'OFF',[]}},'InitialValueBuildCheck9',{{1,'OFF',[]}},'InitialValueBuildCheck10',{{0,'OFF',[]}},'InitialValueBuildCheck11',{{0,'OFF',[]}},'InitialValueBuildCheck12',{{0,'OFF',[]}},'InitialValueBuildCheck13',{{0,'OFF',[]}},'InitialValueBuildCheck14',{{0,'OFF',[]}},'InitialValueBuildCheck15',{{0,'OFF',[]}},'InitialValueBuildCheck16',{{0,'OFF',[]}},'TermValueBuildCheck1',{{0,'OFF',[]}},'TermValueBuildCheck2',{{0,'OFF',[]}},'TermValueBuildCheck3',{{0,'OFF',[]}},'TermValueBuildCheck4',{{0,'OFF',[]}},'TermValueBuildCheck5',{{0,'OFF',[]}},'TermValueBuildCheck6',{{0,'OFF',[]}},'TermValueBuildCheck7',{{0,'OFF',[]}},'TermValueBuildCheck8',{{0,'OFF',[]}},'TermValueBuildCheck9',{{0,'OFF',[]}},'TermValueBuildCheck10',{{0,'OFF',[]}},'TermValueBuildCheck11',{{0,'OFF',[]}},'TermValueBuildCheck12',{{0,'OFF',[]}},'TermValueBuildCheck13',{{0,'OFF',[]}},'TermValueBuildCheck14',{{0,'OFF',[]}},'TermValueBuildCheck15',{{0,'OFF',[]}},'TermValueBuildCheck16',{{0,'OFF',[]}})  RTISFcnParameters=struct('ChannelNo','int16','ChannelNumOf','int16','InitialValue1','double','InitialValue2','double','InitialValue3','double','InitialValue4','double','InitialValue5','double','InitialValue6','double','InitialValue7','double','InitialValue8','double','InitialValue9','double','InitialValue10','double','InitialValue11','double','InitialValue12','double','InitialValue13','double','InitialValue14','double','InitialValue15','double','InitialValue16','double','OutputMode','int16','TermValue1','double','TermValue2','double','TermValue3','double','TermValue4','double','TermValue5','double','TermValue6','double','TermValue7','double','TermValue8','double','TermValue9','double','TermValue10','double','TermValue11','double','TermValue12','double','TermValue13','double','TermValue14','double','TermValue15','double','TermValue16','double','EnableTermMode','int16','TLCFileName','char')  RTIBlockParaDefault=struct('ChannelNo',1,'ChannelNumOf',1,'InitialValue1',0,'InitialValue2',0,'InitialValue3',0,'InitialValue4',0,'InitialValue5',0,'InitialValue6',0,'InitialValue7',0,'InitialValue8',0,'InitialValue9',0,'InitialValue10',0,'InitialValue11',0,'InitialValue12',0,'InitialValue13',0,'InitialValue14',0,'InitialValue15',0,'InitialValue16',0,'OutputMode',ones(1,16),'TermValue1',0,'TermValue2',0,'TermValue3',0,'TermValue4',0,'TermValue5',0,'TermValue6',0,'TermValue7',0,'TermValue8',0,'TermValue9',0,'TermValue10',0,'TermValue11',0,'TermValue12',0,'TermValue13',0,'TermValue14',0,'TermValue15',0,'TermValue16',0,'EnableTermMode',0,'TLCFileName','rti120xdac_c1_dac','InitialValueBuildCheck1',0,'InitialValueBuildCheck2',0,'InitialValueBuildCheck3',0,'InitialValueBuildCheck4',0,'InitialValueBuildCheck5',0,'InitialValueBuildCheck6',0,'InitialValueBuildCheck7',0,'InitialValueBuildCheck8',0,'InitialValueBuildCheck9',0,'InitialValueBuildCheck10',0,'InitialValueBuildCheck11',0,'InitialValueBuildCheck12',0,'InitialValueBuildCheck13',0,'InitialValueBuildCheck14',0,'InitialValueBuildCheck15',0,'InitialValueBuildCheck16',0,'TermValueBuildCheck1',0,'TermValueBuildCheck2',0,'TermValueBuildCheck3',0,'TermValueBuildCheck4',0,'TermValueBuildCheck5',0,'TermValueBuildCheck6',0,'TermValueBuildCheck7',0,'TermValueBuildCheck8',0,'TermValueBuildCheck9',0,'TermValueBuildCheck10',0,'TermValueBuildCheck11',0,'TermValueBuildCheck12',0,'TermValueBuildCheck13',0,'TermValueBuildCheck14',0,'TermValueBuildCheck15',0,'TermValueBuildCheck16',0)
  SineSweep_TMS : Subsystem
  Sinus_TMS : Subsystem
  Sum : Sum  Inputs=+-|
  Sum1 : Sum  Inputs=+-|
  Sum2 : Sum  Inputs=+-|
  Switch Excitation_TMS : Constant  Value=Switch_excit
  TMS_Command : Subsystem
  Terminator{,1,5..9} (7 alike) : Terminator  Commented=on
  Terminator{10,12..23} (13 alike) : Terminator
  F_shaker : Outport  SignalName=F_Shaker  VectorParamsAs1DForOutWhenUnconnected=off
  wires:
  Current monitoring/3(PMA3_current) -> Terminator14/1
  PMA Accelerometers/1(acc1) -> Terminator1/1
  PMA Accelerometers/2(acc2) -> Terminator5/1
  PMA Accelerometers/4(acc4) -> Terminator7/1
  PMA Accelerometers/5(acc5) -> Terminator8/1
  PMA Accelerometers/6(acc6) -> Terminator9/1
  PMA Accelerometers/3(acc3) -> Terminator6/1
  Current monitoring/2(PMA2_current) -> Terminator12/1
  Current monitoring/1(PMA1_current) -> Terminator13/1
  Current monitoring/4(PMA4_current) -> Terminator15/1
  Current monitoring/5(PMA5_current) -> Terminator16/1
  Current monitoring/6(PMA6_current) -> Terminator17/1
  Saturation1/1 -> Micromega PMA2/1, Micromega PMA1/1
  Saturation/1 -> Micromega PMA4/1, Micromega PMA3/1
  Saturation2/1 -> Micromega PMA5/1, Micromega PMA6/1
  Payload Accelerometers/1(Payload_acc1) -> Sum/2, Harmonics Estimator/1(Acc_x)
  Payload Accelerometers/2(Payload_acc2) -> Harmonics Estimator/2(Acc_y), Sum1/2
  Payload Accelerometers/3(Payload_acc3) -> Sum2/2, Harmonics Estimator/3(Acc_z)
  Controller/2(y_command) -> Saturation1/1
  Controller/3(z_command) -> Saturation2/1
  PRBS_TMS/1 -> Multiport Switch2/4
  Saturation_TMS/1 -> TMS_Command/1(In1)
  OFF_TMS/1 -> Multiport Switch2/5
  Sinus_TMS/1(Signal) -> Multiport Switch2/2
  Multiport Switch2/1 -> Saturation_TMS/1
  Switch Excitation_TMS/1 -> Multiport Switch2/1
  SineSweep_TMS/1(Signal) -> Multiport Switch2/3
  PCB208C01/1 -> Force_measure/1(In1)
  Force_measure/1(Excitation [N]) -> F_shaker/1
  Reference_x/1 -> Sum/1
  Reference_y/1 -> Sum1/1
  Harmonics Estimator/1(Peak_freqs_x) -> Terminator/1
  Sum1/1 -> Controller/2(In2)
  Sum2/1 -> Controller/3(In3)
  Sum/1 -> Controller/1(In1)
  Reference_z/1 -> Sum2/1
  Clock/1(Timestamp) -> Terminator10/1
  IMU/5(Gyro_Y (rad/s)) -> Terminator22/1
  IMU/4(Gyro_X (rad/s)) -> Terminator21/1
  IMU/1(Acc_X (m/s^2)) -> Terminator19/1
  IMU/6(Gyro_Z (rad/s)) -> Terminator23/1
  IMU/2(Acc_Y (m/s^2)) -> Terminator18/1
  IMU/3(Acc_Z (m/s^2)) -> Terminator20/1
  TMS_Command/1(Command (V)) -> MATLAB Function/1(exc)
  MATLAB Function/1(u_exc_cmd) -> Controller/4(u_exc_cmd)
  Id on or dist/1 -> MATLAB Function/2(Exc_Route)
  MATLAB Function/2(u_exc_dist) -> Shaker TMS_2007E/1
  Controller/1(x_command) -> Saturation/1
